simulink model "UAV_Hover_Sim"  (R2026b)
settings: Solver=VariableStepAuto  StopTime=15
undefined symbols (not defined in the file): quad_m, W
libraries: slpidlib x1, aerolibanimutils x1, uavutilslib x1
settings Model: Creator=Aorus PC  LastModifiedBy=Ninad
settings OptimizationCC: ReuseModelBlockBuffer=off
settings DebuggingCC: MergeDetectMultiDrivingBlocksExec=none  UnderspecifiedInitializationDetection=Classic
settings ModelReferenceCC: PropagateSignalLabelsOutOfModel=off

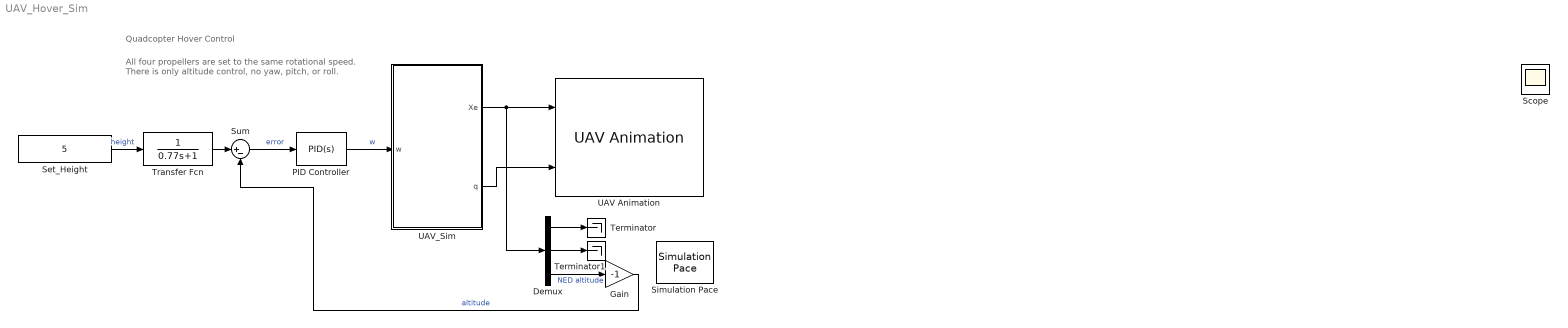
== system UAV_Hover_Sim ==
  note: All four propellers are set to the same rotational speed.
      | There is only altitude control, no yaw, pitch, or roll.
  note: Quadcopter Hover Control
  Demux : Demux  Outputs=3
  Gain : Gain  Gain=-1
  PID Controller : slpidlib/PID Controller  Controller=PID  Form=Parallel  TimeDomain=Continuous-time  UseExternalTs=off  SampleTime=-1  IntegratorMethod=Forward Euler  FilterMethod=Forward Euler  ControllerParametersSource=internal  P=1034  I=448  UseKiTs=off  D=795  UseExternalDerivativeSource=off  N=50  UseFilter=on  TunerSelectOption=Transfer Function Based (PID Tuner App)  InitialConditionSource=internal  InitialConditionForIntegrator=4000  InitialConditionForFilter=0  DifferentiatorICPrevScaledInput=0  ExternalReset=none  TrackingMode=off  Kt=1  LimitOutput=on  SatLimitsSource=internal  UpperSaturationLimit=10000  LowerSaturationLimit=0  LinearizeAsGain=on  AntiWindupMode=back-calculation  Kb=1  LimitIntegrator=on  UpperIntegratorSaturationLimit=10000  LowerIntegratorSaturationLimit=0  POutMin=[]  POutMax=[]  IOutMin=[]  IOutMax=[]  DOutMin=[]  DOutMax=[]  NOutMin=[]  NOutMax=[]  SumOutMin=[]  SumOutMax=[]  SaturationOutMin=[]  SaturationOutMax=[]  PParamMin=[]  PParamMax=[]  IParamMin=[]  IParamMax=[]  DParamMin=[]  DParamMax=[]  NParamMin=[]  NParamMax=[]  KbParamMin=[]  KbParamMax=[]  KtParamMin=[]  KtParamMax=[]  KbOutMin=[]  KbOutMax=[]  KtOutMin=[]  KtOutMax=[]  IntegratorOutMin=[]  IntegratorOutMax=[]  FilterOutMin=[]  FilterOutMax=[]  SumI1OutMin=[]  SumI1OutMax=[]  SumI2OutMin=[]  SumI2OutMax=[]  SumI3OutMin=[]  SumI3OutMax=[]  SumI4OutMin=[]  SumI4OutMax=[]  SumDOutMin=[]  SumDOutMax=[]  DifferentiatorOutMin=[]  DifferentiatorOutMax=[]  FilterDiffOutCoefMin=[]  FilterDiffOutCoefMax=[]  ReciprocalOutMin=[]  ReciprocalOutMax=[]  SumDenOutMin=[]  SumDenOutMax=[]  SumNumOutMin=[]  SumNumOutMax=[]  DivideOutMin=[]  DivideOutMax=[]  UdiffTsProdOutMin=[]  UdiffTsProdOutMax=[]  NTsProdOutMin=[]  NTsProdOutMax=[]  UintegralTsProdOutMin=[]  UintegralTsProdOutMax=[]  UngainTsProdOutMin=[]  UngainTsProdOutMax=[]  ClampingZeroOutDataTypeStr=Inherit: Inherit via back propagation  ClampingZeroOutMin=[]  ClampingZeroOutMax=[]  FilterDenConstantOutDataTypeStr=Inherit: Inherit via back propagation  FilterDenConstantOutMin=[]  FilterDenConstantOutMax=[]  PCopyOutDataTypeStr=Inherit: Inherit via back propagation  PCopyOutMin=[]  PCopyOutMax=[]  NCopyOutDataTypeStr=Inherit: Inherit via back propagation  NCopyOutMin=[]  NCopyOutMax=[]  IntegratorContinuousStateAttributes=''  IntegratorStateMustResolveToSignalObject=off  IntegratorRTWStateStorageClass=Auto  FilterContinuousStateAttributes=''  FilterStateMustResolveToSignalObject=off  FilterRTWStateStorageClass=Auto  ParallelPVariant=InternalParameters  IdealPVariant=Disabled  IVariant=InternalParameters  DVariant=InternalParameters  IntegratorVariant=Continuous  SatVariant=Enabled  AWVariant=BackCalculation  PCopyVariant=Disabled  TRVariant=Disabled  FdbkBlocksVariant=Forward  IdealPFdbkVariant=Disabled  SatFdbkVariant=Disabled  DerivativeFilterVariant=ContFilter  NVariant=InternalParameters  NCopyVariant=Disabled  FilterICVariant=InternalICsFilter  IntegratorICVariant=InternalICs  ExternalResetVariant=Disabled  TRSumVariant=Passthrough  SumFdbkVariant=Disabled  SumVariant=Sum_PID  TsampFilterVariant=InternalTs  TsampNgainVariant=Passthrough  TsampIntegralVariant=Disabled_SignalSpec  ExternalSaturationOutDataTypeStr=Inherit: Same as second input  DerivativeSourceVariant=ErrorSignal  PreIntVariant=InternalPreInt
  Set_Height : Constant  Value=5
  Simulation Pace : aerolibanimutils/Simulation Pace  SimulationPace=1  SleepMode=Auto  OutputPaceError=off  SampleTime=1/30
  Sum : Sum  Inputs=|+-
  Terminator : Terminator
  Terminator1 : Terminator
  Transfer Fcn : TransferFcn  Denominator=[0.77 1]
  UAV Animation : uavutilslib/UAV Animation  NumUAV=1  DynamicUAVConfig=off  UAVType=Multirotor  UAVSize=4  UAVColor=[1 0 0]  UAVTrajectoryAlpha=1  AlwaysShowAnimation=on  AxisLimits=[-Inf Inf;-Inf Inf;-Inf Inf]  TrajectoryBufferSize=100000  InertialZDirection=Down  RotationFormat=Quaternion  DrawMarkers=off  SampleTime=-1
  UAV_Sim : Subsystem
  Scope : Scope
      settings: TimeSpan=20  ActiveDisplayYMinimum=-0.30204491741871653  ActiveDisplayYMaximum=8.4923327241828872  YLabel=Altitude (m)
  wires:
  UAV_Sim/1(Xe) -> Demux/1, UAV Animation/1
  UAV_Sim/2(q) -> UAV Animation/2
  Demux/1 -> Terminator/1
  Demux/2 -> Terminator1/1
  Gain/1 -> Sum/2  "altitude"
  Demux/3 -> Gain/1  "NED altitude"
  PID Controller/1 -> UAV_Sim/1(w)  "w"
  Sum/1 -> PID Controller/1  "error"
  Set_Height/1 -> Transfer Fcn/1  "height"
  Transfer Fcn/1 -> Sum/1

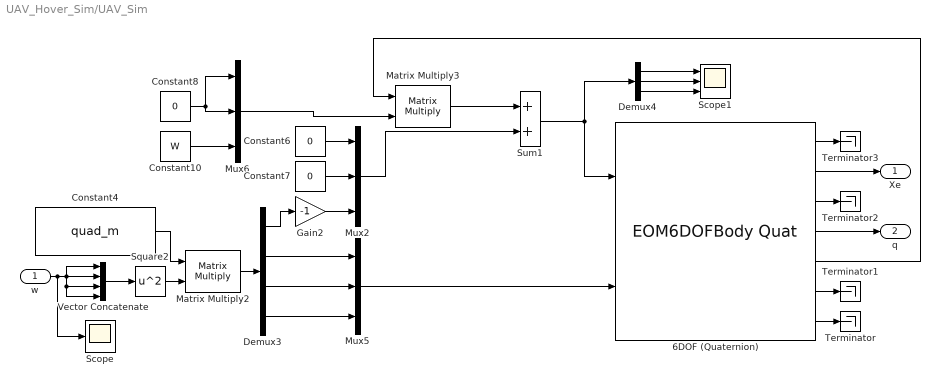
== system UAV_Hover_Sim/UAV_Sim ==
  w : Inport
  6DOF (Quaternion) : EOM6DOFBodyQuat
  Constant10 : Constant  Value=W
  Constant4 : Constant  Value=quad_m
  Constant6 : Constant  Value=0
  Constant7 : Constant  Value=0
  Constant8 : Constant  Value=0
  Demux3 : Demux
  Demux4 : Demux  Outputs=3
  Gain2 : Gain  Gain=-1
  Matrix Multiply2 : Product  Multiplication=Matrix(*)
  Matrix Multiply3 : Product  Multiplication=Matrix(*)
  Mux2 : Mux  Inputs=3
  Mux5 : Mux  Inputs=3
  Mux6 : Mux  Inputs=3
  Scope : Scope
      settings: ActiveDisplayYMinimum=186.55806393636044  ActiveDisplayYMaximum=11090.382437340404
  Scope1 : Scope  NumInputPorts=3
      settings: ActiveDisplayYMinimum=-1  ActiveDisplayYMaximum=1  DataLoggingVariableName=ScopeData2
  Square2 : Math  Operator=square
  Sum1 : Sum
  Terminator{,1..3} (4 alike) : Terminator
  Vector Concatenate : Concatenate  NumInputs=4
  Xe : Outport
  q : Outport  Port=2
  wires:
  Mux2/1 -> Sum1/2
  Matrix Multiply3/1 -> Sum1/1
  Demux4/1 -> Scope1/1
  Mux6/1 -> Matrix Multiply3/2
  Constant10/1 -> Mux6/3
  Sum1/1 -> 6DOF (Quaternion)/1, Demux4/1
  Demux4/2 -> Scope1/2
  Constant4/1 -> Matrix Multiply2/1
  Demux3/1 -> Gain2/1
  Square2/1 -> Matrix Multiply2/2
  Matrix Multiply2/1 -> Demux3/1
  Demux3/2 -> Mux5/1
  Demux3/3 -> Mux5/2
  Demux3/4 -> Mux5/3
  Constant8/1 -> Mux6/2, Mux6/1
  Constant6/1 -> Mux2/1
  Constant7/1 -> Mux2/2
  Gain2/1 -> Mux2/3
  Demux4/3 -> Scope1/3
  w/1 -> Scope/1, Vector Concatenate/4, Vector Concatenate/3, Vector Concatenate/1, Vector Concatenate/2
  6DOF (Quaternion)/4 -> q/1
  6DOF (Quaternion)/5 -> Matrix Multiply3/1
  6DOF (Quaternion)/2 -> Xe/1
  Vector Concatenate/1 -> Square2/1
  Mux5/1 -> 6DOF (Quaternion)/2
  6DOF (Quaternion)/7 -> Terminator/1
  6DOF (Quaternion)/6 -> Terminator1/1
  6DOF (Quaternion)/3 -> Terminator2/1
  6DOF (Quaternion)/1 -> Terminator3/1
